simulink model "IEEE33BusTestSystem_Instantaneous"  (R2019a)
settings: Solver=FixedStepAuto  StartTime=0.0  StopTime=0.2  FixedStep=50e-6  RelTol=1e-3
libraries: powerlib x141, powerlib_meascontrol x2
(part 2 of 3)

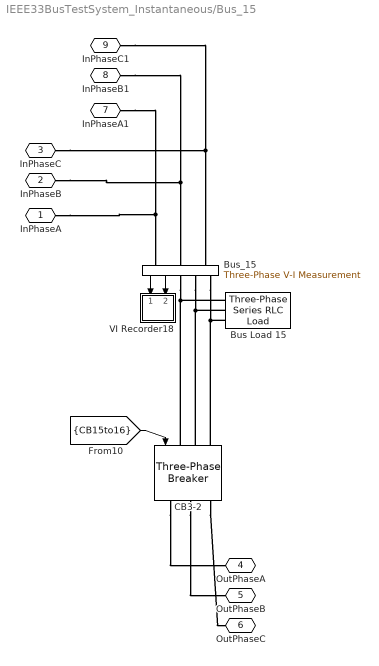
== system IEEE33BusTestSystem_Instantaneous/Bus_15 ==
  Bus Load 15 : powerlib/Elements/Three-Phase Series RLC Load  LConnTagsString=A|B|C  Configuration=Y (grounded)  NominalVoltage=(12660)*0.917215  Vabc=[1e3 1e3 1e3]  Vabcp=[1e3 1e3 1e3]  NominalFrequency=50  UnbalancedPower=off  ActivePower=60e3  InductivePower=10e3  CapacitivePower=0  Pabc=[10e3 9e3 11e3]  QLabc=[100 90 110]  QCabc=[100 90 110]  Pabcp=[10e3 9e3 11e3]  QLabcp=[100 90 110]  QCabcp=[100 90 110]  Measurements=None  LoadType=constant PQ
      settings: SourceProductName=Simscape Electrical
  Bus_15 : powerlib/Measurements/Three-Phase V-I Measurement  VoltageMeasurement=phase-to-phase  SetLabelV=off  LabelV=Vabc  Vpu=off  VpuLL=off  CurrentMeasurement=yes  SetLabelI=off  LabelI=Iabc  Ipu=off  Pbase=100e6  Vbase=500e3  OutputType=Complex  PhasorSimulation=off  PSBequivalent=0
      settings: SourceProductName=Simscape Electrical
  CB3-2 : powerlib/Elements/Three-Phase Breaker  InitialState=open  SwitchA=on  SwitchB=on  SwitchC=on  SwitchTimes="[1/60  5/60]"  External=on  BreakerResistance=0.01  SnubberResistance=1e6  SnubberCapacitance=inf  Measurements=None
      settings: SourceProductName=Simscape Electrical
  VI Recorder18 : Subsystem
  InPhaseA : PMIOPort  Side=Left
  InPhaseB : PMIOPort  Port=2  Side=Left
  InPhaseC : PMIOPort  Port=3  Side=Left
  OutPhaseA : PMIOPort  Port=4  Side=Right
  OutPhaseB : PMIOPort  Port=5  Side=Right
  OutPhaseC : PMIOPort  Port=6  Side=Right
  InPhaseA1 : PMIOPort  Port=7  Side=Left
  InPhaseB1 : PMIOPort  Port=8  Side=Left
  InPhaseC1 : PMIOPort  Port=9  Side=Left
  wires:
  [CB15to16] -> CB3-2/1
  Bus_15/1 -> VI Recorder18/1(Vrec)
  Bus_15/2 -> VI Recorder18/2(Irec)
  connections:
  Bus Load 15/LConn1 -- CB3-2/LConn1 -- Bus_15/RConn1
  CB3-2/RConn3 -- OutPhaseC/RConn1
  Bus Load 15/LConn2 -- CB3-2/LConn2 -- Bus_15/RConn2
  Bus Load 15/LConn3 -- CB3-2/LConn3 -- Bus_15/RConn3
  CB3-2/RConn1 -- OutPhaseA/RConn1
  CB3-2/RConn2 -- OutPhaseB/RConn1
  InPhaseA1/RConn1 -- InPhaseA/RConn1 -- Bus_15/LConn1
  InPhaseB1/RConn1 -- InPhaseB/RConn1 -- Bus_15/LConn2
  InPhaseC1/RConn1 -- InPhaseC/RConn1 -- Bus_15/LConn3

== system IEEE33BusTestSystem_Instantaneous/Bus_16 ==
  Bus Load 16 : powerlib/Elements/Three-Phase Series RLC Load  LConnTagsString=A|B|C  Configuration=Y (grounded)  NominalVoltage=(12660)*0.915849  Vabc=[1e3 1e3 1e3]  Vabcp=[1e3 1e3 1e3]  NominalFrequency=50  UnbalancedPower=off  ActivePower=60e3  InductivePower=20e3  CapacitivePower=0  Pabc=[10e3 9e3 11e3]  QLabc=[100 90 110]  QCabc=[100 90 110]  Pabcp=[10e3 9e3 11e3]  QLabcp=[100 90 110]  QCabcp=[100 90 110]  Measurements=None  LoadType=constant PQ
      settings: SourceProductName=Simscape Electrical
  Bus_16 : powerlib/Measurements/Three-Phase V-I Measurement  VoltageMeasurement=phase-to-phase  SetLabelV=off  LabelV=Vabc  Vpu=off  VpuLL=off  CurrentMeasurement=yes  SetLabelI=off  LabelI=Iabc  Ipu=off  Pbase=100e6  Vbase=500e3  OutputType=Complex  PhasorSimulation=off  PSBequivalent=0
      settings: SourceProductName=Simscape Electrical
  CB3-2 : powerlib/Elements/Three-Phase Breaker  InitialState=open  SwitchA=on  SwitchB=on  SwitchC=on  SwitchTimes="[1/60  5/60]"  External=on  BreakerResistance=0.01  SnubberResistance=1e6  SnubberCapacitance=inf  Measurements=None
      settings: SourceProductName=Simscape Electrical
  VI Recorder19 : Subsystem
  InPhaseA : PMIOPort  Side=Left
  InPhaseB : PMIOPort  Port=2  Side=Left
  InPhaseC : PMIOPort  Port=3  Side=Left
  OutPhaseA : PMIOPort  Port=4  Side=Right
  OutPhaseB : PMIOPort  Port=5  Side=Right
  OutPhaseC : PMIOPort  Port=6  Side=Right
  wires:
  [CB16to17] -> CB3-2/1
  Bus_16/1 -> VI Recorder19/1(Vrec)
  Bus_16/2 -> VI Recorder19/2(Irec)
  connections:
  Bus_16/RConn1 -- CB3-2/LConn1 -- Bus Load 16/LConn1
  CB3-2/RConn3 -- OutPhaseC/RConn1
  Bus Load 16/LConn2 -- CB3-2/LConn2 -- Bus_16/RConn2
  Bus Load 16/LConn3 -- CB3-2/LConn3 -- Bus_16/RConn3
  CB3-2/RConn1 -- OutPhaseA/RConn1
  CB3-2/RConn2 -- OutPhaseB/RConn1
  InPhaseC/RConn1 -- Bus_16/LConn3
  InPhaseB/RConn1 -- Bus_16/LConn2
  InPhaseA/RConn1 -- Bus_16/LConn1

== system IEEE33BusTestSystem_Instantaneous/Bus_17 ==
  Bus Load 17 : powerlib/Elements/Three-Phase Series RLC Load  LConnTagsString=A|B|C  Configuration=Y (grounded)  NominalVoltage=(12660)*0.913826  Vabc=[1e3 1e3 1e3]  Vabcp=[1e3 1e3 1e3]  NominalFrequency=50  UnbalancedPower=off  ActivePower=60e3  InductivePower=20e3  CapacitivePower=0  Pabc=[10e3 9e3 11e3]  QLabc=[100 90 110]  QCabc=[100 90 110]  Pabcp=[10e3 9e3 11e3]  QLabcp=[100 90 110]  QCabcp=[100 90 110]  Measurements=None  LoadType=constant PQ
      settings: SourceProductName=Simscape Electrical
  Bus_17 : powerlib/Measurements/Three-Phase V-I Measurement  VoltageMeasurement=phase-to-phase  SetLabelV=off  LabelV=Vabc  Vpu=off  VpuLL=off  CurrentMeasurement=yes  SetLabelI=off  LabelI=Iabc  Ipu=off  Pbase=100e6  Vbase=500e3  OutputType=Complex  PhasorSimulation=off  PSBequivalent=0
      settings: SourceProductName=Simscape Electrical
  CB3-2 : powerlib/Elements/Three-Phase Breaker  InitialState=open  SwitchA=on  SwitchB=on  SwitchC=on  SwitchTimes="[1/60  5/60]"  External=on  BreakerResistance=0.01  SnubberResistance=1e6  SnubberCapacitance=inf  Measurements=None
      settings: SourceProductName=Simscape Electrical
  VI Recorder20 : Subsystem
  InPhaseA : PMIOPort  Side=Left
  InPhaseB : PMIOPort  Port=2  Side=Left
  InPhaseC : PMIOPort  Port=3  Side=Left
  OutPhaseA : PMIOPort  Port=4  Side=Right
  OutPhaseB : PMIOPort  Port=5  Side=Right
  OutPhaseC : PMIOPort  Port=6  Side=Right
  wires:
  [CB17to18] -> CB3-2/1
  Bus_17/2 -> VI Recorder20/2(Irec)
  Bus_17/1 -> VI Recorder20/1(Vrec)
  connections:
  Bus_17/RConn1 -- CB3-2/LConn1 -- Bus Load 17/LConn1
  CB3-2/RConn3 -- OutPhaseC/RConn1
  Bus Load 17/LConn2 -- CB3-2/LConn2 -- Bus_17/RConn2
  Bus_17/RConn3 -- CB3-2/LConn3 -- Bus Load 17/LConn3
  CB3-2/RConn1 -- OutPhaseA/RConn1
  CB3-2/RConn2 -- OutPhaseB/RConn1
  InPhaseA/RConn1 -- Bus_17/LConn1
  InPhaseB/RConn1 -- Bus_17/LConn2
  InPhaseC/RConn1 -- Bus_17/LConn3

== system IEEE33BusTestSystem_Instantaneous/Bus_18 ==
  Bus Load 18 : powerlib/Elements/Three-Phase Series RLC Load  LConnTagsString=A|B|C  Configuration=Y (grounded)  NominalVoltage=(12660)*0.91322  Vabc=[1e3 1e3 1e3]  Vabcp=[1e3 1e3 1e3]  NominalFrequency=50  UnbalancedPower=off  ActivePower=90e3  InductivePower=40e3  CapacitivePower=0  Pabc=[10e3 9e3 11e3]  QLabc=[100 90 110]  QCabc=[100 90 110]  Pabcp=[10e3 9e3 11e3]  QLabcp=[100 90 110]  QCabcp=[100 90 110]  Measurements=None  LoadType=constant PQ
      settings: SourceProductName=Simscape Electrical
  Bus_18 : powerlib/Measurements/Three-Phase V-I Measurement  VoltageMeasurement=phase-to-phase  SetLabelV=off  LabelV=Vabc  Vpu=off  VpuLL=off  CurrentMeasurement=yes  SetLabelI=off  LabelI=Iabc  Ipu=off  Pbase=100e6  Vbase=500e3  OutputType=Complex  PhasorSimulation=off  PSBequivalent=0
      settings: SourceProductName=Simscape Electrical
  CB3-2 : powerlib/Elements/Three-Phase Breaker  InitialState=open  SwitchA=on  SwitchB=on  SwitchC=on  SwitchTimes="[1/60  5/60]"  External=on  BreakerResistance=0.01  SnubberResistance=1e6  SnubberCapacitance=inf  Measurements=None
      settings: SourceProductName=Simscape Electrical
  VI Recorder21 : Subsystem
  InPhaseA : PMIOPort  Side=Left
  InPhaseB : PMIOPort  Port=2  Side=Left
  InPhaseC : PMIOPort  Port=3  Side=Left
  OutPhaseA : PMIOPort  Port=4  Side=Right
  OutPhaseB : PMIOPort  Port=5  Side=Right
  OutPhaseC : PMIOPort  Port=6  Side=Right
  wires:
  [CB18to33] -> CB3-2/1
  Bus_18/1 -> VI Recorder21/1(Vrec)
  Bus_18/2 -> VI Recorder21/2(Irec)
  connections:
  Bus_18/RConn1 -- CB3-2/LConn1 -- Bus Load 18/LConn1
  CB3-2/RConn3 -- OutPhaseC/RConn1
  Bus Load 18/LConn2 -- CB3-2/LConn2 -- Bus_18/RConn2
  Bus Load 18/LConn3 -- CB3-2/LConn3 -- Bus_18/RConn3
  CB3-2/RConn1 -- OutPhaseA/RConn1
  CB3-2/RConn2 -- OutPhaseB/RConn1
  InPhaseA/RConn1 -- Bus_18/LConn1
  InPhaseB/RConn1 -- Bus_18/LConn2
  InPhaseC/RConn1 -- Bus_18/LConn3

== system IEEE33BusTestSystem_Instantaneous/Bus_19 ==
  Bus Load 19 : powerlib/Elements/Three-Phase Series RLC Load  LConnTagsString=A|B|C  Configuration=Y (grounded)  NominalVoltage=(12660)*0.996507  Vabc=[1e3 1e3 1e3]  Vabcp=[1e3 1e3 1e3]  NominalFrequency=50  UnbalancedPower=off  ActivePower=90e3  InductivePower=40e3  CapacitivePower=0  Pabc=[10e3 9e3 11e3]  QLabc=[100 90 110]  QCabc=[100 90 110]  Pabcp=[10e3 9e3 11e3]  QLabcp=[100 90 110]  QCabcp=[100 90 110]  Measurements=None  LoadType=constant PQ
      settings: SourceProductName=Simscape Electrical
  Bus_19 : powerlib/Measurements/Three-Phase V-I Measurement  VoltageMeasurement=phase-to-phase  SetLabelV=off  LabelV=Vabc  Vpu=off  VpuLL=off  CurrentMeasurement=yes  SetLabelI=off  LabelI=Iabc  Ipu=off  Pbase=100e6  Vbase=500e3  OutputType=Complex  PhasorSimulation=off  PSBequivalent=0
      settings: SourceProductName=Simscape Electrical
  CB3-2 : powerlib/Elements/Three-Phase Breaker  InitialState=open  SwitchA=on  SwitchB=on  SwitchC=on  SwitchTimes="[1/60  5/60]"  External=on  BreakerResistance=0.01  SnubberResistance=1e6  SnubberCapacitance=inf  Measurements=None
      settings: SourceProductName=Simscape Electrical
  VI Recorder : Subsystem
  InPhaseA : PMIOPort  Side=Left
  InPhaseB : PMIOPort  Port=2  Side=Left
  InPhaseC : PMIOPort  Port=3  Side=Left
  OutPhaseA : PMIOPort  Port=4  Side=Right
  OutPhaseB : PMIOPort  Port=5  Side=Right
  OutPhaseC : PMIOPort  Port=6  Side=Right
  wires:
  [CB19to20] -> CB3-2/1
  Bus_19/2 -> VI Recorder/2(Irec)
  Bus_19/1 -> VI Recorder/1(Vrec)
  connections:
  Bus_19/RConn1 -- CB3-2/LConn1 -- Bus Load 19/LConn1
  CB3-2/RConn3 -- OutPhaseC/RConn1
  Bus Load 19/LConn2 -- CB3-2/LConn2 -- Bus_19/RConn2
  Bus_19/RConn3 -- CB3-2/LConn3 -- Bus Load 19/LConn3
  CB3-2/RConn1 -- OutPhaseA/RConn1
  CB3-2/RConn2 -- OutPhaseB/RConn1
  Bus_19/LConn1 -- InPhaseA/RConn1
  InPhaseB/RConn1 -- Bus_19/LConn2
  InPhaseC/RConn1 -- Bus_19/LConn3

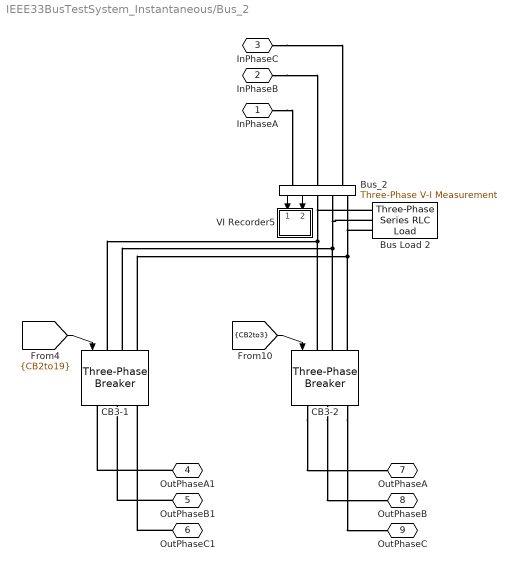
== system IEEE33BusTestSystem_Instantaneous/Bus_2 ==
  Bus Load 2 : powerlib/Elements/Three-Phase Series RLC Load  LConnTagsString=A|B|C  Configuration=Y (grounded)  NominalVoltage=(12660)*0.997035  Vabc=[1e3 1e3 1e3]  Vabcp=[1e3 1e3 1e3]  NominalFrequency=50  UnbalancedPower=off  ActivePower=100e3  InductivePower=60e3  CapacitivePower=0  Pabc=[10e3 9e3 11e3]  QLabc=[100 90 110]  QCabc=[100 90 110]  Pabcp=[10e3 9e3 11e3]  QLabcp=[100 90 110]  QCabcp=[100 90 110]  Measurements=None  LoadType=constant PQ
      settings: SourceProductName=Simscape Electrical
  Bus_2 : powerlib/Measurements/Three-Phase V-I Measurement  VoltageMeasurement=phase-to-phase  SetLabelV=off  LabelV=Vabc  Vpu=off  VpuLL=off  CurrentMeasurement=yes  SetLabelI=off  LabelI=Iabc  Ipu=off  Pbase=100e6  Vbase=500e3  OutputType=Complex  PhasorSimulation=off  PSBequivalent=0
      settings: SourceProductName=Simscape Electrical
  CB3-1 : powerlib/Elements/Three-Phase Breaker  InitialState=open  SwitchA=on  SwitchB=on  SwitchC=on  SwitchTimes="[1/60  5/60]"  External=on  BreakerResistance=0.01  SnubberResistance=1e6  SnubberCapacitance=inf  Measurements=None
      settings: SourceProductName=Simscape Electrical
  CB3-2 : powerlib/Elements/Three-Phase Breaker  InitialState=open  SwitchA=on  SwitchB=on  SwitchC=on  SwitchTimes="[1/60  5/60]"  External=on  BreakerResistance=0.01  SnubberResistance=1e6  SnubberCapacitance=inf  Measurements=None
      settings: SourceProductName=Simscape Electrical
  VI Recorder5 : Subsystem
  InPhaseA : PMIOPort  Side=Left
  InPhaseB : PMIOPort  Port=2  Side=Left
  InPhaseC : PMIOPort  Port=3  Side=Left
  OutPhaseA1 : PMIOPort  Port=4  Side=Right
  OutPhaseB1 : PMIOPort  Port=5  Side=Right
  OutPhaseC1 : PMIOPort  Port=6  Side=Right
  OutPhaseA : PMIOPort  Port=7  Side=Right
  OutPhaseB : PMIOPort  Port=8  Side=Right
  OutPhaseC : PMIOPort  Port=9  Side=Right
  wires:
  [CB2to3] -> CB3-2/1
  Bus_2/2 -> VI Recorder5/2(Irec)
  Bus_2/1 -> VI Recorder5/1(Vrec)
  [CB2to19] -> CB3-1/1
  connections:
  CB3-1/LConn1 -- CB3-2/LConn1 -- Bus Load 2/LConn1 -- Bus_2/RConn1
  CB3-1/LConn2 -- Bus Load 2/LConn2 -- Bus_2/RConn2 -- CB3-2/LConn2
  CB3-1/LConn3 -- Bus Load 2/LConn3 -- Bus_2/RConn3 -- CB3-2/LConn3
  InPhaseC/RConn1 -- Bus_2/LConn3
  InPhaseB/RConn1 -- Bus_2/LConn2
  InPhaseA/RConn1 -- Bus_2/LConn1
  OutPhaseA1/RConn1 -- CB3-1/RConn1
  OutPhaseC1/RConn1 -- CB3-1/RConn3
  OutPhaseB1/RConn1 -- CB3-1/RConn2
  CB3-2/RConn1 -- OutPhaseA/RConn1
  CB3-2/RConn2 -- OutPhaseB/RConn1
  CB3-2/RConn3 -- OutPhaseC/RConn1

== system IEEE33BusTestSystem_Instantaneous/Bus_20 ==
  Bus Load 20 : powerlib/Elements/Three-Phase Series RLC Load  LConnTagsString=A|B|C  Configuration=Y (grounded)  NominalVoltage=(12660)*0.992929  Vabc=[1e3 1e3 1e3]  Vabcp=[1e3 1e3 1e3]  NominalFrequency=50  UnbalancedPower=off  ActivePower=90e3  InductivePower=40e3  CapacitivePower=0  Pabc=[10e3 9e3 11e3]  QLabc=[100 90 110]  QCabc=[100 90 110]  Pabcp=[10e3 9e3 11e3]  QLabcp=[100 90 110]  QCabcp=[100 90 110]  Measurements=None  LoadType=constant PQ
      settings: SourceProductName=Simscape Electrical
  Bus_20 : powerlib/Measurements/Three-Phase V-I Measurement  VoltageMeasurement=phase-to-phase  SetLabelV=off  LabelV=Vabc  Vpu=off  VpuLL=off  CurrentMeasurement=yes  SetLabelI=off  LabelI=Iabc  Ipu=off  Pbase=100e6  Vbase=500e3  OutputType=Complex  PhasorSimulation=off  PSBequivalent=0
      settings: SourceProductName=Simscape Electrical
  CB3-2 : powerlib/Elements/Three-Phase Breaker  InitialState=open  SwitchA=on  SwitchB=on  SwitchC=on  SwitchTimes="[1/60  5/60]"  External=on  BreakerResistance=0.01  SnubberResistance=1e6  SnubberCapacitance=inf  Measurements=None
      settings: SourceProductName=Simscape Electrical
  VI Recorder1 : Subsystem
  InPhaseA : PMIOPort  Side=Left
  InPhaseB : PMIOPort  Port=2  Side=Left
  InPhaseC : PMIOPort  Port=3  Side=Left
  OutPhaseA : PMIOPort  Port=4  Side=Right
  OutPhaseB : PMIOPort  Port=5  Side=Right
  OutPhaseC : PMIOPort  Port=6  Side=Right
  wires:
  [CB20to21] -> CB3-2/1
  Bus_20/1 -> VI Recorder1/1(Vrec)
  Bus_20/2 -> VI Recorder1/2(Irec)
  connections:
  Bus_20/RConn1 -- CB3-2/LConn1 -- Bus Load 20/LConn1
  CB3-2/RConn3 -- OutPhaseC/RConn1
  Bus Load 20/LConn2 -- CB3-2/LConn2 -- Bus_20/RConn2
  Bus_20/RConn3 -- CB3-2/LConn3 -- Bus Load 20/LConn3
  CB3-2/RConn1 -- OutPhaseA/RConn1
  CB3-2/RConn2 -- OutPhaseB/RConn1
  InPhaseA/RConn1 -- Bus_20/LConn1
  InPhaseB/RConn1 -- Bus_20/LConn2
  InPhaseC/RConn1 -- Bus_20/LConn3

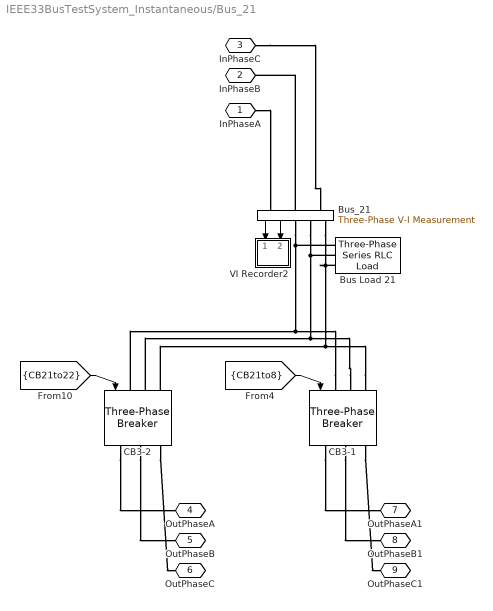
== system IEEE33BusTestSystem_Instantaneous/Bus_21 ==
  Bus Load 21 : powerlib/Elements/Three-Phase Series RLC Load  LConnTagsString=A|B|C  Configuration=Y (grounded)  NominalVoltage=(12660)*0.992224  Vabc=[1e3 1e3 1e3]  Vabcp=[1e3 1e3 1e3]  NominalFrequency=50  UnbalancedPower=off  ActivePower=90e3  InductivePower=40e3  CapacitivePower=0  Pabc=[10e3 9e3 11e3]  QLabc=[100 90 110]  QCabc=[100 90 110]  Pabcp=[10e3 9e3 11e3]  QLabcp=[100 90 110]  QCabcp=[100 90 110]  Measurements=None  LoadType=constant PQ
      settings: SourceProductName=Simscape Electrical
  Bus_21 : powerlib/Measurements/Three-Phase V-I Measurement  VoltageMeasurement=phase-to-phase  SetLabelV=off  LabelV=Vabc  Vpu=off  VpuLL=off  CurrentMeasurement=yes  SetLabelI=off  LabelI=Iabc  Ipu=off  Pbase=100e6  Vbase=500e3  OutputType=Complex  PhasorSimulation=off  PSBequivalent=0
      settings: SourceProductName=Simscape Electrical
  CB3-1 : powerlib/Elements/Three-Phase Breaker  InitialState=open  SwitchA=on  SwitchB=on  SwitchC=on  SwitchTimes="[1/60  5/60]"  External=on  BreakerResistance=0.01  SnubberResistance=1e6  SnubberCapacitance=inf  Measurements=None
      settings: SourceProductName=Simscape Electrical
  CB3-2 : powerlib/Elements/Three-Phase Breaker  InitialState=open  SwitchA=on  SwitchB=on  SwitchC=on  SwitchTimes="[1/60  5/60]"  External=on  BreakerResistance=0.01  SnubberResistance=1e6  SnubberCapacitance=inf  Measurements=None
      settings: SourceProductName=Simscape Electrical
  VI Recorder2 : Subsystem
  InPhaseA : PMIOPort  Side=Left
  InPhaseB : PMIOPort  Port=2  Side=Left
  InPhaseC : PMIOPort  Port=3  Side=Left
  OutPhaseA : PMIOPort  Port=4  Side=Right
  OutPhaseB : PMIOPort  Port=5  Side=Right
  OutPhaseC : PMIOPort  Port=6  Side=Right
  OutPhaseA1 : PMIOPort  Port=7  Side=Right
  OutPhaseB1 : PMIOPort  Port=8  Side=Right
  OutPhaseC1 : PMIOPort  Port=9  Side=Right
  wires:
  [CB21to22] -> CB3-2/1
  Bus_21/2 -> VI Recorder2/2(Irec)
  Bus_21/1 -> VI Recorder2/1(Vrec)
  [CB21to8] -> CB3-1/1
  connections:
  CB3-1/LConn1 -- Bus Load 21/LConn1 -- Bus_21/RConn1 -- CB3-2/LConn1
  CB3-2/RConn3 -- OutPhaseC/RConn1
  CB3-1/LConn2 -- Bus Load 21/LConn2 -- Bus_21/RConn2 -- CB3-2/LConn2
  CB3-1/LConn3 -- Bus_21/RConn3 -- Bus Load 21/LConn3 -- CB3-2/LConn3
  CB3-2/RConn1 -- OutPhaseA/RConn1
  CB3-2/RConn2 -- OutPhaseB/RConn1
  InPhaseA/RConn1 -- Bus_21/LConn1
  Bus_21/LConn2 -- InPhaseB/RConn1
  InPhaseC/RConn1 -- Bus_21/LConn3
  CB3-1/RConn3 -- OutPhaseC1/RConn1
  CB3-1/RConn1 -- OutPhaseA1/RConn1
  CB3-1/RConn2 -- OutPhaseB1/RConn1

== system IEEE33BusTestSystem_Instantaneous/Bus_22 ==
  Bus Load 22 : powerlib/Elements/Three-Phase Series RLC Load  LConnTagsString=A|B|C  Configuration=Y (grounded)  NominalVoltage=(12660)*0.991587  Vabc=[1e3 1e3 1e3]  Vabcp=[1e3 1e3 1e3]  NominalFrequency=50  UnbalancedPower=off  ActivePower=90e3  InductivePower=40e3  CapacitivePower=0  Pabc=[10e3 9e3 11e3]  QLabc=[100 90 110]  QCabc=[100 90 110]  Pabcp=[10e3 9e3 11e3]  QLabcp=[100 90 110]  QCabcp=[100 90 110]  Measurements=None  LoadType=constant PQ
      settings: SourceProductName=Simscape Electrical
  Bus_22 : powerlib/Measurements/Three-Phase V-I Measurement  VoltageMeasurement=phase-to-phase  SetLabelV=off  LabelV=Vabc  Vpu=off  VpuLL=off  CurrentMeasurement=yes  SetLabelI=off  LabelI=Iabc  Ipu=off  Pbase=100e6  Vbase=500e3  OutputType=Complex  PhasorSimulation=off  PSBequivalent=0
      settings: SourceProductName=Simscape Electrical
  CB3-2 : powerlib/Elements/Three-Phase Breaker  InitialState=open  SwitchA=on  SwitchB=on  SwitchC=on  SwitchTimes="[1/60  5/60]"  External=on  BreakerResistance=0.01  SnubberResistance=1e6  SnubberCapacitance=inf  Measurements=None
      settings: SourceProductName=Simscape Electrical
  VI Recorder3 : Subsystem
  InPhaseA : PMIOPort  Side=Left
  InPhaseB : PMIOPort  Port=2  Side=Left
  InPhaseC : PMIOPort  Port=3  Side=Left
  OutPhaseA : PMIOPort  Port=4  Side=Right
  OutPhaseB : PMIOPort  Port=5  Side=Right
  OutPhaseC : PMIOPort  Port=6  Side=Right
  wires:
  [CB22to12] -> CB3-2/1
  Bus_22/2 -> VI Recorder3/2(Irec)
  Bus_22/1 -> VI Recorder3/1(Vrec)
  connections:
  CB3-2/RConn3 -- OutPhaseC/RConn1
  Bus_22/RConn2 -- Bus Load 22/LConn2 -- CB3-2/LConn2
  Bus_22/RConn3 -- Bus Load 22/LConn3 -- CB3-2/LConn3
  CB3-2/RConn1 -- OutPhaseA/RConn1
  CB3-2/RConn2 -- OutPhaseB/RConn1
  Bus Load 22/LConn1 -- CB3-2/LConn1 -- Bus_22/RConn1
  InPhaseA/RConn1 -- Bus_22/LConn1
  InPhaseB/RConn1 -- Bus_22/LConn2
  InPhaseC/RConn1 -- Bus_22/LConn3

== system IEEE33BusTestSystem_Instantaneous/Bus_23 ==
  Bus Load 23 : powerlib/Elements/Three-Phase Series RLC Load  LConnTagsString=A|B|C  Configuration=Y (grounded)  NominalVoltage=(12660)*0.97937  Vabc=[1e3 1e3 1e3]  Vabcp=[1e3 1e3 1e3]  NominalFrequency=50  UnbalancedPower=off  ActivePower=90e3  InductivePower=50e3  CapacitivePower=0  Pabc=[10e3 9e3 11e3]  QLabc=[100 90 110]  QCabc=[100 90 110]  Pabcp=[10e3 9e3 11e3]  QLabcp=[100 90 110]  QCabcp=[100 90 110]  Measurements=None  LoadType=constant PQ
      settings: SourceProductName=Simscape Electrical
  Bus_23 : powerlib/Measurements/Three-Phase V-I Measurement  VoltageMeasurement=phase-to-phase  SetLabelV=off  LabelV=Vabc  Vpu=off  VpuLL=off  CurrentMeasurement=yes  SetLabelI=off  LabelI=Iabc  Ipu=off  Pbase=100e6  Vbase=500e3  OutputType=Complex  PhasorSimulation=off  PSBequivalent=0
      settings: SourceProductName=Simscape Electrical
  CB3-2 : powerlib/Elements/Three-Phase Breaker  InitialState=open  SwitchA=on  SwitchB=on  SwitchC=on  SwitchTimes="[1/60  5/60]"  External=on  BreakerResistance=0.01  SnubberResistance=1e6  SnubberCapacitance=inf  Measurements=None
      settings: SourceProductName=Simscape Electrical
  VI Recorder32 : Subsystem
  InPhaseA : PMIOPort  Side=Left
  InPhaseB : PMIOPort  Port=2  Side=Left
  InPhaseC : PMIOPort  Port=3  Side=Left
  OutPhaseA : PMIOPort  Port=4  Side=Right
  OutPhaseB : PMIOPort  Port=5  Side=Right
  OutPhaseC : PMIOPort  Port=6  Side=Right
  wires:
  Bus_23/2 -> VI Recorder32/2(Irec)
  Bus_23/1 -> VI Recorder32/1(Vrec)
  [CB23to24] -> CB3-2/1
  connections:
  Bus_23/RConn1 -- CB3-2/LConn1 -- Bus Load 23/LConn1
  CB3-2/RConn3 -- OutPhaseC/RConn1
  Bus Load 23/LConn2 -- CB3-2/LConn2 -- Bus_23/RConn2
  Bus Load 23/LConn3 -- CB3-2/LConn3 -- Bus_23/RConn3
  CB3-2/RConn1 -- OutPhaseA/RConn1
  CB3-2/RConn2 -- OutPhaseB/RConn1
  InPhaseA/RConn1 -- Bus_23/LConn1
  InPhaseB/RConn1 -- Bus_23/LConn2
  InPhaseC/RConn1 -- Bus_23/LConn3

== system IEEE33BusTestSystem_Instantaneous/Bus_24 ==
  Bus Load 24 : powerlib/Elements/Three-Phase Series RLC Load  LConnTagsString=A|B|C  Configuration=Y (grounded)  NominalVoltage=(12660)*0.9727  Vabc=[1e3 1e3 1e3]  Vabcp=[1e3 1e3 1e3]  NominalFrequency=50  UnbalancedPower=off  ActivePower=420e3  InductivePower=200e3  CapacitivePower=0  Pabc=[10e3 9e3 11e3]  QLabc=[100 90 110]  QCabc=[100 90 110]  Pabcp=[10e3 9e3 11e3]  QLabcp=[100 90 110]  QCabcp=[100 90 110]  Measurements=None  LoadType=constant PQ
      settings: SourceProductName=Simscape Electrical
  Bus_24 : powerlib/Measurements/Three-Phase V-I Measurement  VoltageMeasurement=phase-to-phase  SetLabelV=off  LabelV=Vabc  Vpu=off  VpuLL=off  CurrentMeasurement=yes  SetLabelI=off  LabelI=Iabc  Ipu=off  Pbase=100e6  Vbase=500e3  OutputType=Complex  PhasorSimulation=off  PSBequivalent=0
      settings: SourceProductName=Simscape Electrical
  CB3-2 : powerlib/Elements/Three-Phase Breaker  InitialState=open  SwitchA=on  SwitchB=on  SwitchC=on  SwitchTimes="[1/60  5/60]"  External=on  BreakerResistance=0.01  SnubberResistance=1e6  SnubberCapacitance=inf  Measurements=None
      settings: SourceProductName=Simscape Electrical
  VI Recorder31 : Subsystem
  InPhaseA : PMIOPort  Side=Left
  InPhaseB : PMIOPort  Port=2  Side=Left
  InPhaseC : PMIOPort  Port=3  Side=Left
  OutPhaseA : PMIOPort  Port=4  Side=Right
  OutPhaseB : PMIOPort  Port=5  Side=Right
  OutPhaseC : PMIOPort  Port=6  Side=Right
  wires:
  Bus_24/1 -> VI Recorder31/1(Vrec)
  Bus_24/2 -> VI Recorder31/2(Irec)
  [CB24to25] -> CB3-2/1
  connections:
  Bus_24/RConn1 -- CB3-2/LConn1 -- Bus Load 24/LConn1
  CB3-2/RConn3 -- OutPhaseC/RConn1
  Bus Load 24/LConn2 -- CB3-2/LConn2 -- Bus_24/RConn2
  Bus Load 24/LConn3 -- CB3-2/LConn3 -- Bus_24/RConn3
  CB3-2/RConn1 -- OutPhaseA/RConn1
  CB3-2/RConn2 -- OutPhaseB/RConn1
  InPhaseA/RConn1 -- Bus_24/LConn1
  InPhaseB/RConn1 -- Bus_24/LConn2
  InPhaseC/RConn1 -- Bus_24/LConn3

== system IEEE33BusTestSystem_Instantaneous/Bus_25 ==
  Bus Load 25 : powerlib/Elements/Three-Phase Series RLC Load  LConnTagsString=A|B|C  Configuration=Y (grounded)  NominalVoltage=(12660)*0.969375  Vabc=[1e3 1e3 1e3]  Vabcp=[1e3 1e3 1e3]  NominalFrequency=50  UnbalancedPower=off  ActivePower=420e3  InductivePower=200e3  CapacitivePower=0  Pabc=[10e3 9e3 11e3]  QLabc=[100 90 110]  QCabc=[100 90 110]  Pabcp=[10e3 9e3 11e3]  QLabcp=[100 90 110]  QCabcp=[100 90 110]  Measurements=None  LoadType=constant PQ
      settings: SourceProductName=Simscape Electrical
  Bus_25 : powerlib/Measurements/Three-Phase V-I Measurement  VoltageMeasurement=phase-to-phase  SetLabelV=off  LabelV=Vabc  Vpu=off  VpuLL=off  CurrentMeasurement=yes  SetLabelI=off  LabelI=Iabc  Ipu=off  Pbase=100e6  Vbase=500e3  OutputType=Complex  PhasorSimulation=off  PSBequivalent=0
      settings: SourceProductName=Simscape Electrical
  CB3-2 : powerlib/Elements/Three-Phase Breaker  InitialState=open  SwitchA=on  SwitchB=on  SwitchC=on  SwitchTimes="[1/60  5/60]"  External=on  BreakerResistance=0.01  SnubberResistance=1e6  SnubberCapacitance=inf  Measurements=None
      settings: SourceProductName=Simscape Electrical
  VI Recorder30 : Subsystem
  InPhaseA : PMIOPort  Side=Left
  InPhaseB : PMIOPort  Port=2  Side=Left
  InPhaseC : PMIOPort  Port=3  Side=Left
  OutPhaseA : PMIOPort  Port=4  Side=Right
  OutPhaseB : PMIOPort  Port=5  Side=Right
  OutPhaseC : PMIOPort  Port=6  Side=Right
  wires:
  Bus_25/2 -> VI Recorder30/2(Irec)
  Bus_25/1 -> VI Recorder30/1(Vrec)
  [CB25to29] -> CB3-2/1
  connections:
  Bus_25/RConn1 -- CB3-2/LConn1 -- Bus Load 25/LConn1
  CB3-2/RConn3 -- OutPhaseC/RConn1
  Bus Load 25/LConn2 -- CB3-2/LConn2 -- Bus_25/RConn2
  Bus_25/RConn3 -- CB3-2/LConn3 -- Bus Load 25/LConn3
  CB3-2/RConn1 -- OutPhaseA/RConn1
  CB3-2/RConn2 -- OutPhaseB/RConn1
  InPhaseB/RConn1 -- Bus_25/LConn2
  InPhaseA/RConn1 -- Bus_25/LConn1
  InPhaseC/RConn1 -- Bus_25/LConn3

== system IEEE33BusTestSystem_Instantaneous/Bus_26 ==
  Bus Load 26 : powerlib/Elements/Three-Phase Series RLC Load  LConnTagsString=A|B|C  Configuration=Y (grounded)  NominalVoltage=(12660)*0.947798  Vabc=[1e3 1e3 1e3]  Vabcp=[1e3 1e3 1e3]  NominalFrequency=50  UnbalancedPower=off  ActivePower=60e3  InductivePower=25e3  CapacitivePower=0  Pabc=[10e3 9e3 11e3]  QLabc=[100 90 110]  QCabc=[100 90 110]  Pabcp=[10e3 9e3 11e3]  QLabcp=[100 90 110]  QCabcp=[100 90 110]  Measurements=None  LoadType=constant PQ
      settings: SourceProductName=Simscape Electrical
  Bus_26 : powerlib/Measurements/Three-Phase V-I Measurement  VoltageMeasurement=phase-to-phase  SetLabelV=off  LabelV=Vabc  Vpu=off  VpuLL=off  CurrentMeasurement=yes  SetLabelI=off  LabelI=Iabc  Ipu=off  Pbase=100e6  Vbase=500e3  OutputType=Complex  PhasorSimulation=off  PSBequivalent=0
      settings: SourceProductName=Simscape Electrical
  CB3-2 : powerlib/Elements/Three-Phase Breaker  InitialState=open  SwitchA=on  SwitchB=on  SwitchC=on  SwitchTimes="[1/60  5/60]"  External=on  BreakerResistance=0.01  SnubberResistance=1e6  SnubberCapacitance=inf  Measurements=None
      settings: SourceProductName=Simscape Electrical
  VI Recorder22 : Subsystem
  InPhaseA : PMIOPort  Side=Left
  InPhaseB : PMIOPort  Port=2  Side=Left
  InPhaseC : PMIOPort  Port=3  Side=Left
  OutPhaseA : PMIOPort  Port=4  Side=Right
  OutPhaseB : PMIOPort  Port=5  Side=Right
  OutPhaseC : PMIOPort  Port=6  Side=Right
  wires:
  Bus_26/2 -> VI Recorder22/2(Irec)
  Bus_26/1 -> VI Recorder22/1(Vrec)
  [CB26to27] -> CB3-2/1
  connections:
  CB3-2/RConn3 -- OutPhaseC/RConn1
  Bus Load 26/LConn2 -- CB3-2/LConn2 -- Bus_26/RConn2
  Bus_26/RConn3 -- CB3-2/LConn3 -- Bus Load 26/LConn3
  CB3-2/RConn1 -- OutPhaseA/RConn1
  CB3-2/RConn2 -- OutPhaseB/RConn1
  Bus_26/RConn1 -- CB3-2/LConn1 -- Bus Load 26/LConn1
  InPhaseA/RConn1 -- Bus_26/LConn1
  InPhaseB/RConn1 -- Bus_26/LConn2
  InPhaseC/RConn1 -- Bus_26/LConn3

== system IEEE33BusTestSystem_Instantaneous/Bus_27 ==
  Bus Load 27 : powerlib/Elements/Three-Phase Series RLC Load  LConnTagsString=A|B|C  Configuration=Y (grounded)  NominalVoltage=(12660)*0.945238  Vabc=[1e3 1e3 1e3]  Vabcp=[1e3 1e3 1e3]  NominalFrequency=50  UnbalancedPower=off  ActivePower=60e3  InductivePower=25e3  CapacitivePower=0  Pabc=[10e3 9e3 11e3]  QLabc=[100 90 110]  QCabc=[100 90 110]  Pabcp=[10e3 9e3 11e3]  QLabcp=[100 90 110]  QCabcp=[100 90 110]  Measurements=None  LoadType=constant PQ
      settings: SourceProductName=Simscape Electrical
  Bus_27 : powerlib/Measurements/Three-Phase V-I Measurement  VoltageMeasurement=phase-to-phase  SetLabelV=off  LabelV=Vabc  Vpu=off  VpuLL=off  CurrentMeasurement=yes  SetLabelI=off  LabelI=Iabc  Ipu=off  Pbase=100e6  Vbase=500e3  OutputType=Complex  PhasorSimulation=off  PSBequivalent=0
      settings: SourceProductName=Simscape Electrical
  CB3-2 : powerlib/Elements/Three-Phase Breaker  InitialState=open  SwitchA=on  SwitchB=on  SwitchC=on  SwitchTimes="[1/60  5/60]"  External=on  BreakerResistance=0.01  SnubberResistance=1e6  SnubberCapacitance=inf  Measurements=None
      settings: SourceProductName=Simscape Electrical
  VI Recorder23 : Subsystem
  InPhaseA : PMIOPort  Side=Left
  InPhaseB : PMIOPort  Port=2  Side=Left
  InPhaseC : PMIOPort  Port=3  Side=Left
  OutPhaseA : PMIOPort  Port=4  Side=Right
  OutPhaseB : PMIOPort  Port=5  Side=Right
  OutPhaseC : PMIOPort  Port=6  Side=Right
  wires:
  Bus_27/1 -> VI Recorder23/1(Vrec)
  Bus_27/2 -> VI Recorder23/2(Irec)
  [CB27to28] -> CB3-2/1
  connections:
  CB3-2/LConn1 -- Bus Load 27/LConn1 -- Bus_27/RConn1
  CB3-2/RConn3 -- OutPhaseC/RConn1
  CB3-2/LConn2 -- Bus Load 27/LConn2 -- Bus_27/RConn2
  Bus_27/RConn3 -- Bus Load 27/LConn3 -- CB3-2/LConn3
  CB3-2/RConn1 -- OutPhaseA/RConn1
  CB3-2/RConn2 -- OutPhaseB/RConn1
  InPhaseA/RConn1 -- Bus_27/LConn1
  InPhaseB/RConn1 -- Bus_27/LConn2
  InPhaseC/RConn1 -- Bus_27/LConn3

== system IEEE33BusTestSystem_Instantaneous/Bus_28 ==
  Bus Load 28 : powerlib/Elements/Three-Phase Series RLC Load  LConnTagsString=A|B|C  Configuration=Y (grounded)  NominalVoltage=(12660)*0.933818  Vabc=[1e3 1e3 1e3]  Vabcp=[1e3 1e3 1e3]  NominalFrequency=50  UnbalancedPower=off  ActivePower=60e3  InductivePower=20e3  CapacitivePower=0  Pabc=[10e3 9e3 11e3]  QLabc=[100 90 110]  QCabc=[100 90 110]  Pabcp=[10e3 9e3 11e3]  QLabcp=[100 90 110]  QCabcp=[100 90 110]  Measurements=None  LoadType=constant PQ
      settings: SourceProductName=Simscape Electrical
  Bus_28 : powerlib/Measurements/Three-Phase V-I Measurement  VoltageMeasurement=phase-to-phase  SetLabelV=off  LabelV=Vabc  Vpu=off  VpuLL=off  CurrentMeasurement=yes  SetLabelI=off  LabelI=Iabc  Ipu=off  Pbase=100e6  Vbase=500e3  OutputType=Complex  PhasorSimulation=off  PSBequivalent=0
      settings: SourceProductName=Simscape Electrical
  CB3-2 : powerlib/Elements/Three-Phase Breaker  InitialState=open  SwitchA=on  SwitchB=on  SwitchC=on  SwitchTimes="[1/60  5/60]"  External=on  BreakerResistance=0.01  SnubberResistance=1e6  SnubberCapacitance=inf  Measurements=None
      settings: SourceProductName=Simscape Electrical
  VI Recorder24 : Subsystem
  InPhaseA : PMIOPort  Side=Left
  InPhaseB : PMIOPort  Port=2  Side=Left
  InPhaseC : PMIOPort  Port=3  Side=Left
  OutPhaseA : PMIOPort  Port=4  Side=Right
  OutPhaseB : PMIOPort  Port=5  Side=Right
  OutPhaseC : PMIOPort  Port=6  Side=Right
  wires:
  Bus_28/2 -> VI Recorder24/2(Irec)
  Bus_28/1 -> VI Recorder24/1(Vrec)
  [CB28to29] -> CB3-2/1
  connections:
  Bus Load 28/LConn1 -- CB3-2/LConn1 -- Bus_28/RConn1
  CB3-2/RConn3 -- OutPhaseC/RConn1
  Bus Load 28/LConn2 -- CB3-2/LConn2 -- Bus_28/RConn2
  Bus Load 28/LConn3 -- CB3-2/LConn3 -- Bus_28/RConn3
  CB3-2/RConn1 -- OutPhaseA/RConn1
  CB3-2/RConn2 -- OutPhaseB/RConn1
  InPhaseA/RConn1 -- Bus_28/LConn1
  InPhaseB/RConn1 -- Bus_28/LConn2
  InPhaseC/RConn1 -- Bus_28/LConn3

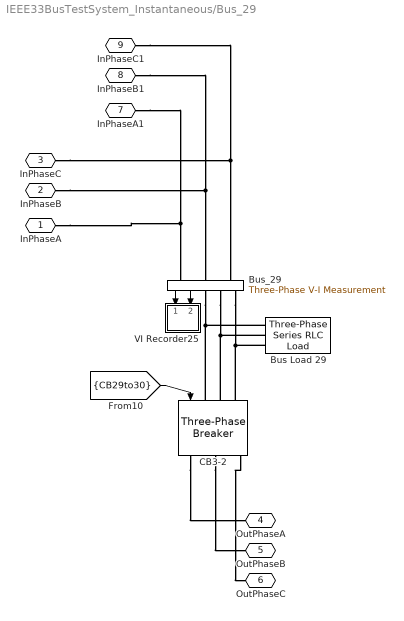
== system IEEE33BusTestSystem_Instantaneous/Bus_29 ==
  Bus Load 29 : powerlib/Elements/Three-Phase Series RLC Load  LConnTagsString=A|B|C  Configuration=Y (grounded)  NominalVoltage=(12660)*0.925614  Vabc=[1e3 1e3 1e3]  Vabcp=[1e3 1e3 1e3]  NominalFrequency=50  UnbalancedPower=off  ActivePower=120e3  InductivePower=70e3  CapacitivePower=0  Pabc=[10e3 9e3 11e3]  QLabc=[100 90 110]  QCabc=[100 90 110]  Pabcp=[10e3 9e3 11e3]  QLabcp=[100 90 110]  QCabcp=[100 90 110]  Measurements=None  LoadType=constant PQ
      settings: SourceProductName=Simscape Electrical
  Bus_29 : powerlib/Measurements/Three-Phase V-I Measurement  VoltageMeasurement=phase-to-phase  SetLabelV=off  LabelV=Vabc  Vpu=off  VpuLL=off  CurrentMeasurement=yes  SetLabelI=off  LabelI=Iabc  Ipu=off  Pbase=100e6  Vbase=500e3  OutputType=Complex  PhasorSimulation=off  PSBequivalent=0
      settings: SourceProductName=Simscape Electrical
  CB3-2 : powerlib/Elements/Three-Phase Breaker  InitialState=open  SwitchA=on  SwitchB=on  SwitchC=on  SwitchTimes="[1/60  5/60]"  External=on  BreakerResistance=0.01  SnubberResistance=1e6  SnubberCapacitance=inf  Measurements=None
      settings: SourceProductName=Simscape Electrical
  VI Recorder25 : Subsystem
  InPhaseA : PMIOPort  Side=Left
  InPhaseB : PMIOPort  Port=2  Side=Left
  InPhaseC : PMIOPort  Port=3  Side=Left
  OutPhaseA : PMIOPort  Port=4  Side=Right
  OutPhaseB : PMIOPort  Port=5  Side=Right
  OutPhaseC : PMIOPort  Port=6  Side=Right
  InPhaseA1 : PMIOPort  Port=7  Side=Left
  InPhaseB1 : PMIOPort  Port=8  Side=Left
  InPhaseC1 : PMIOPort  Port=9  Side=Left
  wires:
  Bus_29/1 -> VI Recorder25/1(Vrec)
  Bus_29/2 -> VI Recorder25/2(Irec)
  [CB29to30] -> CB3-2/1
  connections:
  Bus_29/RConn1 -- CB3-2/LConn1 -- Bus Load 29/LConn1
  CB3-2/RConn3 -- OutPhaseC/RConn1
  Bus Load 29/LConn2 -- CB3-2/LConn2 -- Bus_29/RConn2
  Bus Load 29/LConn3 -- CB3-2/LConn3 -- Bus_29/RConn3
  CB3-2/RConn1 -- OutPhaseA/RConn1
  CB3-2/RConn2 -- OutPhaseB/RConn1
  InPhaseB1/RConn1 -- InPhaseB/RConn1 -- Bus_29/LConn2
  InPhaseA1/RConn1 -- InPhaseA/RConn1 -- Bus_29/LConn1
  InPhaseC1/RConn1 -- InPhaseC/RConn1 -- Bus_29/LConn3

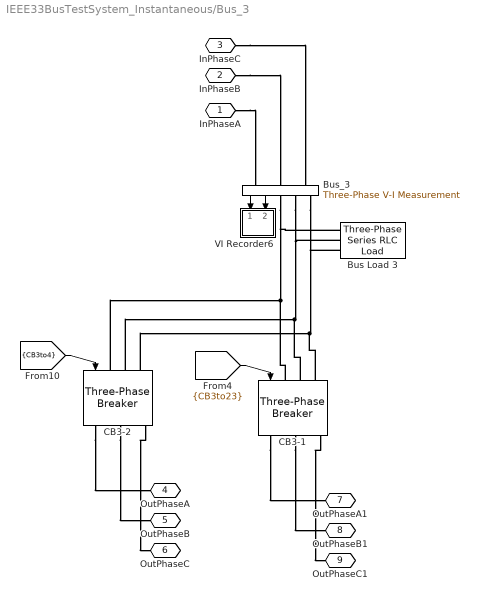
== system IEEE33BusTestSystem_Instantaneous/Bus_3 ==
  Bus Load 3 : powerlib/Elements/Three-Phase Series RLC Load  LConnTagsString=A|B|C  Configuration=Y (grounded)  NominalVoltage=(12660)*0.982955  Vabc=[1e3 1e3 1e3]  Vabcp=[1e3 1e3 1e3]  NominalFrequency=50  UnbalancedPower=off  ActivePower=90e3  InductivePower=40e3  CapacitivePower=0  Pabc=[10e3 9e3 11e3]  QLabc=[100 90 110]  QCabc=[100 90 110]  Pabcp=[10e3 9e3 11e3]  QLabcp=[100 90 110]  QCabcp=[100 90 110]  Measurements=None  LoadType=constant PQ
      settings: SourceProductName=Simscape Electrical
  Bus_3 : powerlib/Measurements/Three-Phase V-I Measurement  VoltageMeasurement=phase-to-phase  SetLabelV=off  LabelV=Vabc  Vpu=off  VpuLL=off  CurrentMeasurement=yes  SetLabelI=off  LabelI=Iabc  Ipu=off  Pbase=100e6  Vbase=500e3  OutputType=Complex  PhasorSimulation=off  PSBequivalent=0
      settings: SourceProductName=Simscape Electrical
  CB3-1 : powerlib/Elements/Three-Phase Breaker  InitialState=open  SwitchA=on  SwitchB=on  SwitchC=on  SwitchTimes="[1/60  5/60]"  External=on  BreakerResistance=0.01  SnubberResistance=1e6  SnubberCapacitance=inf  Measurements=None
      settings: SourceProductName=Simscape Electrical
  CB3-2 : powerlib/Elements/Three-Phase Breaker  InitialState=open  SwitchA=on  SwitchB=on  SwitchC=on  SwitchTimes="[1/60  5/60]"  External=on  BreakerResistance=0.01  SnubberResistance=1e6  SnubberCapacitance=inf  Measurements=None
      settings: SourceProductName=Simscape Electrical
  VI Recorder6 : Subsystem
  InPhaseA : PMIOPort  Side=Left
  InPhaseB : PMIOPort  Port=2  Side=Left
  InPhaseC : PMIOPort  Port=3  Side=Left
  OutPhaseA : PMIOPort  Port=4  Side=Right
  OutPhaseB : PMIOPort  Port=5  Side=Right
  OutPhaseC : PMIOPort  Port=6  Side=Right
  OutPhaseA1 : PMIOPort  Port=7  Side=Right
  OutPhaseB1 : PMIOPort  Port=8  Side=Right
  OutPhaseC1 : PMIOPort  Port=9  Side=Right
  wires:
  Bus_3/2 -> VI Recorder6/2(Irec)
  Bus_3/1 -> VI Recorder6/1(Vrec)
  [CB3to4] -> CB3-2/1
  [CB3to23] -> CB3-1/1
  connections:
  CB3-2/LConn1 -- CB3-1/LConn1 -- Bus Load 3/LConn1 -- Bus_3/RConn1
  CB3-2/RConn3 -- OutPhaseC/RConn1
  CB3-1/LConn2 -- Bus Load 3/LConn2 -- Bus_3/RConn2 -- CB3-2/LConn2
  CB3-1/LConn3 -- Bus_3/RConn3 -- Bus Load 3/LConn3 -- CB3-2/LConn3
  CB3-2/RConn1 -- OutPhaseA/RConn1
  CB3-2/RConn2 -- OutPhaseB/RConn1
  CB3-1/RConn3 -- OutPhaseC1/RConn1
  CB3-1/RConn1 -- OutPhaseA1/RConn1
  CB3-1/RConn2 -- OutPhaseB1/RConn1
  InPhaseA/RConn1 -- Bus_3/LConn1
  InPhaseB/RConn1 -- Bus_3/LConn2
  InPhaseC/RConn1 -- Bus_3/LConn3

== system IEEE33BusTestSystem_Instantaneous/Bus_30 ==
  Bus Load 30 : powerlib/Elements/Three-Phase Series RLC Load  LConnTagsString=A|B|C  Configuration=Y (grounded)  NominalVoltage=(12660)*0.922063  Vabc=[1e3 1e3 1e3]  Vabcp=[1e3 1e3 1e3]  NominalFrequency=50  UnbalancedPower=off  ActivePower=200e3  InductivePower=600e3  CapacitivePower=0  Pabc=[10e3 9e3 11e3]  QLabc=[100 90 110]  QCabc=[100 90 110]  Pabcp=[10e3 9e3 11e3]  QLabcp=[100 90 110]  QCabcp=[100 90 110]  Measurements=None  LoadType=constant PQ
      settings: SourceProductName=Simscape Electrical
  Bus_30 : powerlib/Measurements/Three-Phase V-I Measurement  VoltageMeasurement=phase-to-phase  SetLabelV=off  LabelV=Vabc  Vpu=off  VpuLL=off  CurrentMeasurement=yes  SetLabelI=off  LabelI=Iabc  Ipu=off  Pbase=100e6  Vbase=500e3  OutputType=Complex  PhasorSimulation=off  PSBequivalent=0
      settings: SourceProductName=Simscape Electrical
  CB3-2 : powerlib/Elements/Three-Phase Breaker  InitialState=open  SwitchA=on  SwitchB=on  SwitchC=on  SwitchTimes="[1/60  5/60]"  External=on  BreakerResistance=0.01  SnubberResistance=1e6  SnubberCapacitance=inf  Measurements=None
      settings: SourceProductName=Simscape Electrical
  VI Recorder26 : Subsystem
  InPhaseA : PMIOPort  Side=Left
  InPhaseB : PMIOPort  Port=2  Side=Left
  InPhaseC : PMIOPort  Port=3  Side=Left
  OutPhaseA : PMIOPort  Port=4  Side=Right
  OutPhaseB : PMIOPort  Port=5  Side=Right
  OutPhaseC : PMIOPort  Port=6  Side=Right
  wires:
  Bus_30/1 -> VI Recorder26/1(Vrec)
  Bus_30/2 -> VI Recorder26/2(Irec)
  [CB30to31] -> CB3-2/1
  connections:
  Bus_30/RConn1 -- CB3-2/LConn1 -- Bus Load 30/LConn1
  CB3-2/RConn3 -- OutPhaseC/RConn1
  Bus Load 30/LConn2 -- CB3-2/LConn2 -- Bus_30/RConn2
  Bus Load 30/LConn3 -- CB3-2/LConn3 -- Bus_30/RConn3
  CB3-2/RConn1 -- OutPhaseA/RConn1
  CB3-2/RConn2 -- OutPhaseB/RConn1
  InPhaseB/RConn1 -- Bus_30/LConn2
  InPhaseA/RConn1 -- Bus_30/LConn1
  InPhaseC/RConn1 -- Bus_30/LConn3

== system IEEE33BusTestSystem_Instantaneous/Bus_31 ==
  Bus Load 31 : powerlib/Elements/Three-Phase Series RLC Load  LConnTagsString=A|B|C  Configuration=Y (grounded)  NominalVoltage=(12660)*0.917909  Vabc=[1e3 1e3 1e3]  Vabcp=[1e3 1e3 1e3]  NominalFrequency=50  UnbalancedPower=off  ActivePower=150e3  InductivePower=70e3  CapacitivePower=0  Pabc=[10e3 9e3 11e3]  QLabc=[100 90 110]  QCabc=[100 90 110]  Pabcp=[10e3 9e3 11e3]  QLabcp=[100 90 110]  QCabcp=[100 90 110]  Measurements=None  LoadType=constant PQ
      settings: SourceProductName=Simscape Electrical
  Bus_31 : powerlib/Measurements/Three-Phase V-I Measurement  VoltageMeasurement=phase-to-phase  SetLabelV=off  LabelV=Vabc  Vpu=off  VpuLL=off  CurrentMeasurement=yes  SetLabelI=off  LabelI=Iabc  Ipu=off  Pbase=100e6  Vbase=500e3  OutputType=Complex  PhasorSimulation=off  PSBequivalent=0
      settings: SourceProductName=Simscape Electrical
  CB3-2 : powerlib/Elements/Three-Phase Breaker  InitialState=open  SwitchA=on  SwitchB=on  SwitchC=on  SwitchTimes="[1/60  5/60]"  External=on  BreakerResistance=0.01  SnubberResistance=1e6  SnubberCapacitance=inf  Measurements=None
      settings: SourceProductName=Simscape Electrical
  VI Recorder27 : Subsystem
  InPhaseA : PMIOPort  Side=Left
  InPhaseB : PMIOPort  Port=2  Side=Left
  InPhaseC : PMIOPort  Port=3  Side=Left
  OutPhaseA : PMIOPort  Port=4  Side=Right
  OutPhaseB : PMIOPort  Port=5  Side=Right
  OutPhaseC : PMIOPort  Port=6  Side=Right
  wires:
  Bus_31/2 -> VI Recorder27/2(Irec)
  Bus_31/1 -> VI Recorder27/1(Vrec)
  [CB31to32] -> CB3-2/1
  connections:
  Bus_31/RConn1 -- CB3-2/LConn1 -- Bus Load 31/LConn1
  CB3-2/RConn3 -- OutPhaseC/RConn1
  Bus Load 31/LConn2 -- CB3-2/LConn2 -- Bus_31/RConn2
  Bus Load 31/LConn3 -- CB3-2/LConn3 -- Bus_31/RConn3
  CB3-2/RConn1 -- OutPhaseA/RConn1
  CB3-2/RConn2 -- OutPhaseB/RConn1
  InPhaseA/RConn1 -- Bus_31/LConn1
  Bus_31/LConn2 -- InPhaseB/RConn1
  InPhaseC/RConn1 -- Bus_31/LConn3

== system IEEE33BusTestSystem_Instantaneous/Bus_32 ==
  Bus Load 32 : powerlib/Elements/Three-Phase Series RLC Load  LConnTagsString=A|B|C  Configuration=Y (grounded)  NominalVoltage=(12660)*0.916995  Vabc=[1e3 1e3 1e3]  Vabcp=[1e3 1e3 1e3]  NominalFrequency=50  UnbalancedPower=off  ActivePower=210e3  InductivePower=100e3  CapacitivePower=0  Pabc=[10e3 9e3 11e3]  QLabc=[100 90 110]  QCabc=[100 90 110]  Pabcp=[10e3 9e3 11e3]  QLabcp=[100 90 110]  QCabcp=[100 90 110]  Measurements=None  LoadType=constant PQ
      settings: SourceProductName=Simscape Electrical
  Bus_32 : powerlib/Measurements/Three-Phase V-I Measurement  VoltageMeasurement=phase-to-phase  SetLabelV=off  LabelV=Vabc  Vpu=off  VpuLL=off  CurrentMeasurement=yes  SetLabelI=off  LabelI=Iabc  Ipu=off  Pbase=100e6  Vbase=500e3  OutputType=Complex  PhasorSimulation=off  PSBequivalent=0
      settings: SourceProductName=Simscape Electrical
  CB3-2 : powerlib/Elements/Three-Phase Breaker  InitialState=open  SwitchA=on  SwitchB=on  SwitchC=on  SwitchTimes="[1/60  5/60]"  External=on  BreakerResistance=0.01  SnubberResistance=1e6  SnubberCapacitance=inf  Measurements=None
      settings: SourceProductName=Simscape Electrical
  VI Recorder28 : Subsystem
  InPhaseA : PMIOPort  Side=Left
  InPhaseB : PMIOPort  Port=2  Side=Left
  InPhaseC : PMIOPort  Port=3  Side=Left
  OutPhaseA : PMIOPort  Port=4  Side=Right
  OutPhaseB : PMIOPort  Port=5  Side=Right
  OutPhaseC : PMIOPort  Port=6  Side=Right
  wires:
  Bus_32/2 -> VI Recorder28/2(Irec)
  Bus_32/1 -> VI Recorder28/1(Vrec)
  [CB32to33] -> CB3-2/1
  connections:
  Bus_32/RConn1 -- CB3-2/LConn1 -- Bus Load 32/LConn1
  CB3-2/RConn3 -- OutPhaseC/RConn1
  Bus Load 32/LConn2 -- CB3-2/LConn2 -- Bus_32/RConn2
  Bus_32/RConn3 -- Bus Load 32/LConn3 -- CB3-2/LConn3
  CB3-2/RConn1 -- OutPhaseA/RConn1
  CB3-2/RConn2 -- OutPhaseB/RConn1
  InPhaseA/RConn1 -- Bus_32/LConn1
  InPhaseB/RConn1 -- Bus_32/LConn2
  InPhaseC/RConn1 -- Bus_32/LConn3

== system IEEE33BusTestSystem_Instantaneous/Bus_33 ==
  Bus Load 33 : powerlib/Elements/Three-Phase Series RLC Load  LConnTagsString=A|B|C  Configuration=Y (grounded)  NominalVoltage=(12660)*0.916712  Vabc=[1e3 1e3 1e3]  Vabcp=[1e3 1e3 1e3]  NominalFrequency=50  UnbalancedPower=off  ActivePower=60e3  InductivePower=40e3  CapacitivePower=0  Pabc=[10e3 9e3 11e3]  QLabc=[100 90 110]  QCabc=[100 90 110]  Pabcp=[10e3 9e3 11e3]  QLabcp=[100 90 110]  QCabcp=[100 90 110]  Measurements=None  LoadType=constant PQ
      settings: SourceProductName=Simscape Electrical
  Bus_33 : powerlib/Measurements/Three-Phase V-I Measurement  VoltageMeasurement=phase-to-phase  SetLabelV=off  LabelV=Vabc  Vpu=off  VpuLL=off  CurrentMeasurement=yes  SetLabelI=off  LabelI=Iabc  Ipu=off  Pbase=100e6  Vbase=500e3  OutputType=Complex  PhasorSimulation=off  PSBequivalent=0
      settings: SourceProductName=Simscape Electrical
  VI Recorder29 : Subsystem
  InPhaseA : PMIOPort  Side=Left
  InPhaseB : PMIOPort  Port=2  Side=Left
  InPhaseC : PMIOPort  Port=3  Side=Left
  OutPhaseA : PMIOPort  Port=4  Side=Right
  OutPhaseB : PMIOPort  Port=5  Side=Right
  OutPhaseC : PMIOPort  Port=6  Side=Right
  wires:
  Bus_33/2 -> VI Recorder29/2(Irec)
  Bus_33/1 -> VI Recorder29/1(Vrec)
  connections:
  Bus Load 33/LConn1 -- Bus_33/RConn1 -- OutPhaseA/RConn1
  Bus Load 33/LConn2 -- OutPhaseB/RConn1 -- Bus_33/RConn2
  Bus_33/RConn3 -- OutPhaseC/RConn1 -- Bus Load 33/LConn3
  InPhaseA/RConn1 -- Bus_33/LConn1
  InPhaseB/RConn1 -- Bus_33/LConn2
  InPhaseC/RConn1 -- Bus_33/LConn3

== system IEEE33BusTestSystem_Instantaneous/Bus_4 ==
  Bus Load 4 : powerlib/Elements/Three-Phase Series RLC Load  LConnTagsString=A|B|C  Configuration=Y (grounded)  NominalVoltage=(12660)*0.975484  Vabc=[1e3 1e3 1e3]  Vabcp=[1e3 1e3 1e3]  NominalFrequency=50  UnbalancedPower=off  ActivePower=120e3  InductivePower=80e3  CapacitivePower=0  Pabc=[10e3 9e3 11e3]  QLabc=[100 90 110]  QCabc=[100 90 110]  Pabcp=[10e3 9e3 11e3]  QLabcp=[100 90 110]  QCabcp=[100 90 110]  Measurements=None  LoadType=constant PQ
      settings: SourceProductName=Simscape Electrical
  Bus_4 : powerlib/Measurements/Three-Phase V-I Measurement  VoltageMeasurement=phase-to-phase  SetLabelV=off  LabelV=Vabc  Vpu=off  VpuLL=off  CurrentMeasurement=yes  SetLabelI=off  LabelI=Iabc  Ipu=off  Pbase=100e6  Vbase=500e3  OutputType=Complex  PhasorSimulation=off  PSBequivalent=0
      settings: SourceProductName=Simscape Electrical
  CB3-2 : powerlib/Elements/Three-Phase Breaker  InitialState=open  SwitchA=on  SwitchB=on  SwitchC=on  SwitchTimes="[1/60  5/60]"  External=on  BreakerResistance=0.01  SnubberResistance=1e6  SnubberCapacitance=inf  Measurements=None
      settings: SourceProductName=Simscape Electrical
  VI Recorder7 : Subsystem
  InPhaseA : PMIOPort  Side=Left
  InPhaseB : PMIOPort  Port=2  Side=Left
  InPhaseC : PMIOPort  Port=3  Side=Left
  OutPhaseA : PMIOPort  Port=4  Side=Right
  OutPhaseB : PMIOPort  Port=5  Side=Right
  OutPhaseC : PMIOPort  Port=6  Side=Right
  wires:
  Bus_4/1 -> VI Recorder7/1(Vrec)
  Bus_4/2 -> VI Recorder7/2(Irec)
  [CB4to5] -> CB3-2/1
  connections:
  Bus_4/RConn1 -- CB3-2/LConn1 -- Bus Load 4/LConn1
  CB3-2/RConn3 -- OutPhaseC/RConn1
  Bus Load 4/LConn2 -- CB3-2/LConn2 -- Bus_4/RConn2
  Bus_4/RConn3 -- CB3-2/LConn3 -- Bus Load 4/LConn3
  CB3-2/RConn1 -- OutPhaseA/RConn1
  CB3-2/RConn2 -- OutPhaseB/RConn1
  InPhaseA/RConn1 -- Bus_4/LConn1
  InPhaseB/RConn1 -- Bus_4/LConn2
  InPhaseC/RConn1 -- Bus_4/LConn3

== system IEEE33BusTestSystem_Instantaneous/Bus_5 ==
  Bus Load 5 : powerlib/Elements/Three-Phase Series RLC Load  LConnTagsString=A|B|C  Configuration=Y (grounded)  NominalVoltage=(12660)*0.968098  Vabc=[1e3 1e3 1e3]  Vabcp=[1e3 1e3 1e3]  NominalFrequency=50  UnbalancedPower=off  ActivePower=60e3  InductivePower=30e3  CapacitivePower=0  Pabc=[10e3 9e3 11e3]  QLabc=[100 90 110]  QCabc=[100 90 110]  Pabcp=[10e3 9e3 11e3]  QLabcp=[100 90 110]  QCabcp=[100 90 110]  Measurements=None  LoadType=constant PQ
      settings: SourceProductName=Simscape Electrical
  Bus_5 : powerlib/Measurements/Three-Phase V-I Measurement  VoltageMeasurement=phase-to-phase  SetLabelV=off  LabelV=Vabc  Vpu=off  VpuLL=off  CurrentMeasurement=yes  SetLabelI=off  LabelI=Iabc  Ipu=off  Pbase=100e6  Vbase=500e3  OutputType=Complex  PhasorSimulation=off  PSBequivalent=0
      settings: SourceProductName=Simscape Electrical
  CB3-2 : powerlib/Elements/Three-Phase Breaker  InitialState=open  SwitchA=on  SwitchB=on  SwitchC=on  SwitchTimes="[1/60  5/60]"  External=on  BreakerResistance=0.01  SnubberResistance=1e6  SnubberCapacitance=inf  Measurements=None
      settings: SourceProductName=Simscape Electrical
  VI Recorder8 : Subsystem
  InPhaseA : PMIOPort  Side=Left
  InPhaseB : PMIOPort  Port=2  Side=Left
  InPhaseC : PMIOPort  Port=3  Side=Left
  OutPhaseA : PMIOPort  Port=4  Side=Right
  OutPhaseB : PMIOPort  Port=5  Side=Right
  OutPhaseC : PMIOPort  Port=6  Side=Right
  wires:
  Bus_5/2 -> VI Recorder8/2(Irec)
  Bus_5/1 -> VI Recorder8/1(Vrec)
  [CB5to6] -> CB3-2/1
  connections:
  Bus Load 5/LConn1 -- CB3-2/LConn1 -- Bus_5/RConn1
  CB3-2/RConn3 -- OutPhaseC/RConn1
  Bus_5/RConn2 -- CB3-2/LConn2 -- Bus Load 5/LConn2
  Bus_5/RConn3 -- CB3-2/LConn3 -- Bus Load 5/LConn3
  CB3-2/RConn1 -- OutPhaseA/RConn1
  CB3-2/RConn2 -- OutPhaseB/RConn1
  InPhaseA/RConn1 -- Bus_5/LConn1
  InPhaseB/RConn1 -- Bus_5/LConn2
  InPhaseC/RConn1 -- Bus_5/LConn3

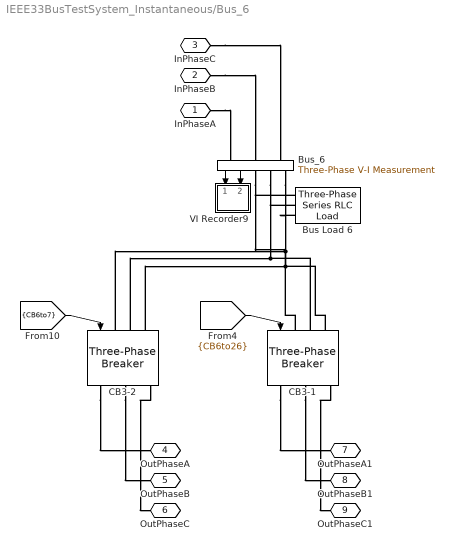
== system IEEE33BusTestSystem_Instantaneous/Bus_6 ==
  Bus Load 6 : powerlib/Elements/Three-Phase Series RLC Load  LConnTagsString=A|B|C  Configuration=Y (grounded)  NominalVoltage=(12660)*0.949724  Vabc=[1e3 1e3 1e3]  Vabcp=[1e3 1e3 1e3]  NominalFrequency=50  UnbalancedPower=off  ActivePower=60e3  InductivePower=20e3  CapacitivePower=0  Pabc=[10e3 9e3 11e3]  QLabc=[100 90 110]  QCabc=[100 90 110]  Pabcp=[10e3 9e3 11e3]  QLabcp=[100 90 110]  QCabcp=[100 90 110]  Measurements=None  LoadType=constant PQ
      settings: SourceProductName=Simscape Electrical
  Bus_6 : powerlib/Measurements/Three-Phase V-I Measurement  VoltageMeasurement=phase-to-phase  SetLabelV=off  LabelV=Vabc  Vpu=off  VpuLL=off  CurrentMeasurement=yes  SetLabelI=off  LabelI=Iabc  Ipu=off  Pbase=100e6  Vbase=500e3  OutputType=Complex  PhasorSimulation=off  PSBequivalent=0
      settings: SourceProductName=Simscape Electrical
  CB3-1 : powerlib/Elements/Three-Phase Breaker  InitialState=open  SwitchA=on  SwitchB=on  SwitchC=on  SwitchTimes="[1/60  5/60]"  External=on  BreakerResistance=0.01  SnubberResistance=1e6  SnubberCapacitance=inf  Measurements=None
      settings: SourceProductName=Simscape Electrical
  CB3-2 : powerlib/Elements/Three-Phase Breaker  InitialState=open  SwitchA=on  SwitchB=on  SwitchC=on  SwitchTimes="[1/60  5/60]"  External=on  BreakerResistance=0.01  SnubberResistance=1e6  SnubberCapacitance=inf  Measurements=None
      settings: SourceProductName=Simscape Electrical
  VI Recorder9 : Subsystem
  InPhaseA : PMIOPort  Side=Left
  InPhaseB : PMIOPort  Port=2  Side=Left
  InPhaseC : PMIOPort  Port=3  Side=Left
  OutPhaseA : PMIOPort  Port=4  Side=Right
  OutPhaseB : PMIOPort  Port=5  Side=Right
  OutPhaseC : PMIOPort  Port=6  Side=Right
  OutPhaseA1 : PMIOPort  Port=7  Side=Right
  OutPhaseB1 : PMIOPort  Port=8  Side=Right
  OutPhaseC1 : PMIOPort  Port=9  Side=Right
  wires:
  Bus_6/1 -> VI Recorder9/1(Vrec)
  Bus_6/2 -> VI Recorder9/2(Irec)
  [CB6to26] -> CB3-1/1
  [CB6to7] -> CB3-2/1
  connections:
  Bus Load 6/LConn1 -- Bus_6/RConn1 -- CB3-2/LConn1 -- CB3-1/LConn1
  CB3-2/RConn3 -- OutPhaseC/RConn1
  Bus Load 6/LConn2 -- Bus_6/RConn2 -- CB3-1/LConn2 -- CB3-2/LConn2
  Bus Load 6/LConn3 -- Bus_6/RConn3 -- CB3-1/LConn3 -- CB3-2/LConn3
  CB3-2/RConn1 -- OutPhaseA/RConn1
  CB3-2/RConn2 -- OutPhaseB/RConn1
  CB3-1/RConn3 -- OutPhaseC1/RConn1
  CB3-1/RConn2 -- OutPhaseB1/RConn1
  CB3-1/RConn1 -- OutPhaseA1/RConn1
  InPhaseA/RConn1 -- Bus_6/LConn1
  InPhaseB/RConn1 -- Bus_6/LConn2
  InPhaseC/RConn1 -- Bus_6/LConn3
